simulink model "pendulo_invertido_lqr"  (R2023b)
settings: Solver=ode45  StartTime=0.0  StopTime=duracion  MaxStep=1e-3  RelTol=1e-8  AbsTol=1e-10
values from neighbouring files (symbols this model uses):
  a = p.a    [INICIAR_PENDULO_SIMULINK.m]
  b_eje = p.b_eje_mecanico    [INICIAR_PENDULO_SIMULINK.m]
  b_m = motor.b_m    [INICIAR_PENDULO_SIMULINK.m]
  b_phi = p.b_phi    [INICIAR_PENDULO_SIMULINK.m]
  b_x = p.b_x    [INICIAR_PENDULO_SIMULINK.m]
  beta_V = motor.beta_V    [INICIAR_PENDULO_SIMULINK.m]
  e_acople = p.e_acople    [INICIAR_PENDULO_SIMULINK.m]
  h = p.h    [INICIAR_PENDULO_SIMULINK.m]
  j = p.j    [INICIAR_PENDULO_SIMULINK.m]
  K = C.K    [INICIAR_PENDULO_SIMULINK.m]
  k = p.k    [INICIAR_PENDULO_SIMULINK.m]
  q0 = [x0; deg2rad(phi0_deg)]    [INICIAR_PENDULO_SIMULINK.m]
  q_punto0 = [v0; omega0]    [INICIAR_PENDULO_SIMULINK.m]
  r = p.r    [INICIAR_PENDULO_SIMULINK.m]
  t_consigna = 2.0    (= 2)    [INICIAR_PENDULO_SIMULINK.m]
  tau_traccion = limite_de_traccion(p)    [INICIAR_PENDULO_SIMULINK.m]    (also in exportar_planta_al_banco.m; ganancias_para_el_firmware.m)
  V_bat = motor.V_bat    [INICIAR_PENDULO_SIMULINK.m]
  x_destino = 0.30    (= 0.3)    [INICIAR_PENDULO_SIMULINK.m]
settings Model: Creator=calde  LastModifiedBy=calde

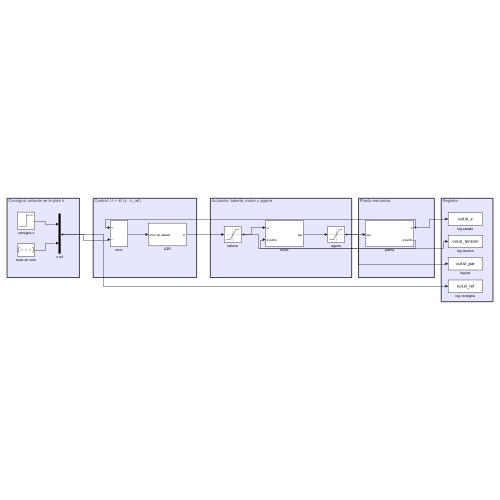
[thumbnail: Simulink's stored preview of the top-level diagram]
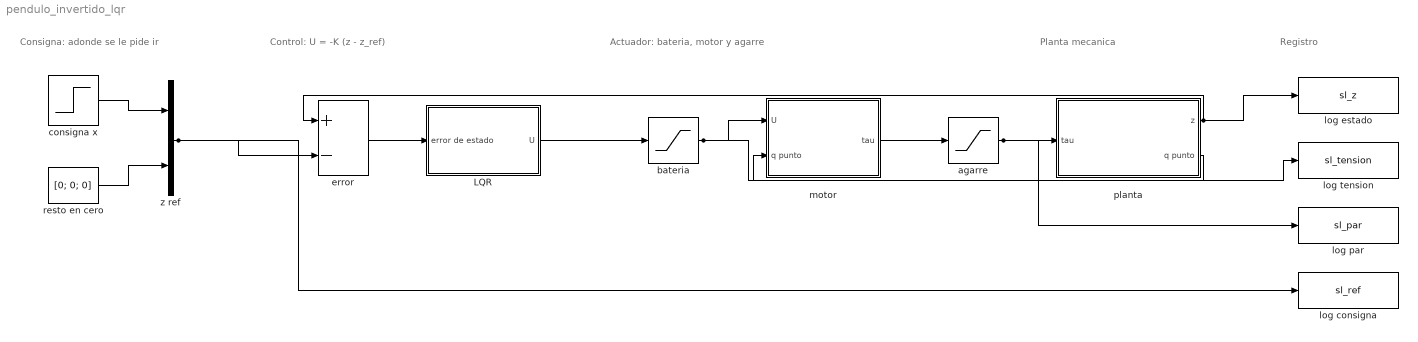
== system pendulo_invertido_lqr ==
  note: Consigna: adonde se le pide ir
  note: Control: U = -K (z - z_ref)
  note: Actuador: bateria, motor y agarre
  note: Planta mecanica
  note: Registro
  LQR : Subsystem
  agarre : Saturate  UpperLimit=tau_traccion  LowerLimit=-tau_traccion
  bateria : Saturate  UpperLimit=V_bat  LowerLimit=-V_bat
  consigna x : Step  Time=t_consigna  After=x_destino  SampleTime=0
  error : Sum  Inputs=+-
  log consigna : ToWorkspace  VariableName=sl_ref  SaveFormat=Structure With Time  SampleTime=-1
  log estado : ToWorkspace  VariableName=sl_z  SaveFormat=Structure With Time  SampleTime=-1
  log par : ToWorkspace  VariableName=sl_par  SaveFormat=Structure With Time  SampleTime=-1
  log tension : ToWorkspace  VariableName=sl_tension  SaveFormat=Structure With Time  SampleTime=-1
  motor : Subsystem
  planta : Subsystem
  resto en cero : Constant  Value=[0; 0; 0]
  z ref : Mux  Inputs=2
  wires:
  consigna x/1 -> z ref/1
  resto en cero/1 -> z ref/2
  z ref/1 -> error/2, log consigna/1
  error/1 -> LQR/1(error de estado)
  LQR/1(U) -> bateria/1
  bateria/1 -> motor/1(U), log tension/1
  motor/1(tau) -> agarre/1
  agarre/1 -> planta/1(tau), log par/1
  planta/1(z) -> error/1, log estado/1
  planta/2(q punto) -> motor/2(q punto)

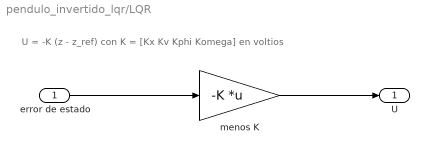
== system pendulo_invertido_lqr/LQR ==
  note: U = -K (z - z_ref) con K = [Kx Kv Kphi Komega] en voltios
  error de estado : Inport
  menos K : Gain  Gain=-K  Multiplication=Matrix(K*u)
  U : Outport
  wires:
  error de estado/1 -> menos K/1
  menos K/1 -> U/1

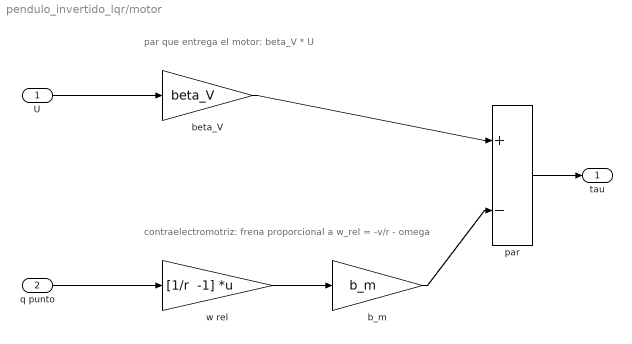
== system pendulo_invertido_lqr/motor ==
  note: par que entrega el motor: beta_V * U
  note: contraelectromotriz: frena proporcional a w_rel = -v/r - omega
  U : Inport
  q punto : Inport  Port=2
  b_m : Gain  Gain=b_m
  beta_V : Gain  Gain=beta_V
  par : Sum  Inputs=+-
  w rel : Gain  Gain="[1/r  -1]"  Multiplication=Matrix(K*u)
  tau : Outport
  wires:
  U/1 -> beta_V/1
  q punto/1 -> w rel/1
  w rel/1 -> b_m/1
  beta_V/1 -> par/1
  b_m/1 -> par/2
  par/1 -> tau/1

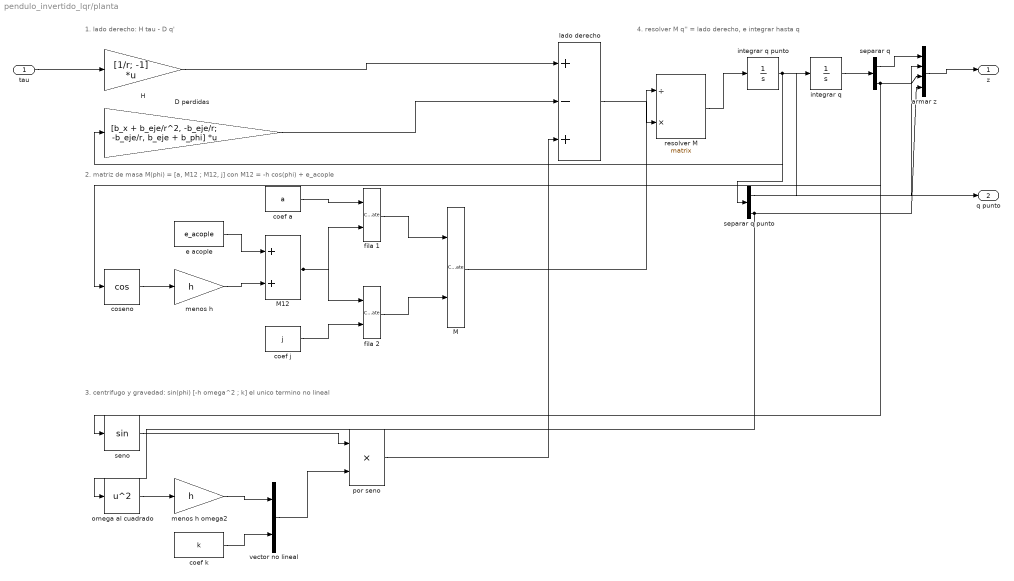
== system pendulo_invertido_lqr/planta ==
  note: 1. lado derecho: H tau - D q'
  note: 2. matriz de masa M(phi) = [a, M12 ; M12, j] con M12 = -h cos(phi) + e_acople
  note: 3. centrifugo y gravedad: sin(phi) [-h omega^2 ; k] el unico termino no lineal
  note: 4. resolver M q'' = lado derecho, e integrar hasta q
  tau : Inport
  D perdidas : Gain  Gain="[b_x + b_eje/r^2,  -b_eje/r;  -b_eje/r,  b_eje + b_phi]"  Multiplication=Matrix(K*u)
  H : Gain  Gain=[1/r; -1]  Multiplication=Matrix(K*u)
  M : Concatenate  Mode=Multidimensional array
  M12 : Sum
  armar z : Mux
  coef a : Constant  Value=a
  coef j : Constant  Value=j
  coef k : Constant  Value=k
  coseno : Trigonometry  Operator=cos
  e acople : Constant  Value=e_acople
  fila 1 : Concatenate  Mode=Multidimensional array  ConcatenateDimension=2
  fila 2 : Concatenate  Mode=Multidimensional array  ConcatenateDimension=2
  integrar q : Integrator  InitialCondition=q0
  integrar q punto : Integrator  InitialCondition=q_punto0
  lado derecho : Sum  Inputs=+-+
  menos h : Gain  Gain=h
  menos h omega2 : Gain  Gain=h
  omega al cuadrado : Math  Operator=square
  por seno : Product
  resolver M : Product  Inputs=/*  Multiplication=Matrix(*)
  seno : Trigonometry
  separar q : Demux  Outputs=2
  separar q punto : Demux  Outputs=2
  vector no lineal : Mux  Inputs=2
  z : Outport
  q punto : Outport  Port=2
  wires:
  resolver M/1 -> integrar q punto/1
  integrar q punto/1 -> integrar q/1, separar q punto/1, q punto/1, D perdidas/1
  integrar q/1 -> separar q/1
  separar q/1 -> armar z/1
  separar q punto/1 -> armar z/2
  separar q/2 -> armar z/3, coseno/1, seno/1
  separar q punto/2 -> armar z/4, omega al cuadrado/1
  armar z/1 -> z/1
  tau/1 -> H/1
  H/1 -> lado derecho/1
  D perdidas/1 -> lado derecho/2
  por seno/1 -> lado derecho/3
  coseno/1 -> menos h/1
  menos h/1 -> M12/2
  e acople/1 -> M12/1
  coef a/1 -> fila 1/1
  M12/1 -> fila 1/2, fila 2/1
  coef j/1 -> fila 2/2
  fila 1/1 -> M/1
  fila 2/1 -> M/2
  omega al cuadrado/1 -> menos h omega2/1
  menos h omega2/1 -> vector no lineal/1
  coef k/1 -> vector no lineal/2
  seno/1 -> por seno/1
  vector no lineal/1 -> por seno/2
  M/1 -> resolver M/1
  lado derecho/1 -> resolver M/2
